simulink model "cable_driven_parallel_robot2022"  (R2022b)
settings: Solver=ode3  StartTime=0.0  StopTime=100  FixedStep=0.01  RelTol=1e-3
values from neighbouring files (symbols this model uses):
  cable_length = 1.2    [Model_Info.m]
  g = 9.81    [Model_Info.m]
  MP_H = 2    [Model_Info.m]
  MP_init_X = 0    [Model_Info.m]
  MP_init_Y = 0    [Model_Info.m]
  MP_init_Z = cable_length + (MP_H/2)    (= 2.2)    [Model_Info.m]
  MP_Ix = (MP_m/12)*(MP_W^2+MP_H^2)    (= 6.66666666667e-05)    [Model_Info.m]
  MP_Iy = (MP_m/12)*(MP_L^2+MP_H^2)    (= 6.66666666667e-05)    [Model_Info.m]
  MP_Iz = (MP_m/12)*(MP_L^2+MP_W^2)    (= 6.66666666667e-05)    [Model_Info.m]
  MP_L = 2    [Model_Info.m]
  MP_m = 0.0001    [Model_Info.m]
  MP_W = 2    [Model_Info.m]
  MR_init_X_L1 = -(MP_L/2)    (= -1)    [Model_Info.m]
  MR_init_X_L2 = (MP_L/2)    (= 1)    [Model_Info.m]
  MR_init_X_L3 = (MP_L/2)    (= 1)    [Model_Info.m]
  MR_init_X_L4 = -(MP_L/2)    (= -1)    [Model_Info.m]
  MR_init_Y_L1 = -(MP_W/2)    (= -1)    [Model_Info.m]
  MR_init_Y_L2 = -(MP_W/2)    (= -1)    [Model_Info.m]
  MR_init_Y_L3 = (MP_W/2)    (= 1)    [Model_Info.m]
  MR_init_Y_L4 = (MP_W/2)    (= 1)    [Model_Info.m]
  MR_init_Yaw_L1 = pi    (= 3.14159265359)    [Model_Info.m]
  MR_init_Yaw_L2 = 0    [Model_Info.m]
  MR_init_Yaw_L3 = 0    [Model_Info.m]
  MR_init_Yaw_L4 = pi    (= 3.14159265359)    [Model_Info.m]
  MR_Jr = (MR_m/12)*(MR_L^2+MR_W^2)    (= 0.333333333333)    [Model_Info.m]
  MR_m = 0.5    [Model_Info.m]
  MR_r = 2    [Model_Info.m]
  MR_WT = 2    [Model_Info.m]
  QR_Ax = 0.25*0    (= 0)    [Model_Info.m]
  QR_Ay = 0.25*0    (= 0)    [Model_Info.m]
  QR_Az = 0.25*0    (= 0)    [Model_Info.m]
  QR_b = 1.14*1e-7    (= 1.14e-07)    [Model_Info.m]
  QR_Ixx = 4.856*1e-3    (= 0.004856)    [Model_Info.m]
  QR_Iyy = 4.856*1e-3    (= 0.004856)    [Model_Info.m]
  QR_Izz = 8.801*1e-3    (= 0.008801)    [Model_Info.m]
  QR_K = 2.980*1e-6    (= 2.98e-06)    [Model_Info.m]
  QR_l = 0.225    [Model_Info.m]
  QR_m = 0.468    [Model_Info.m]
  QR_x0_U1 = -(MP_L/2)    (= -1)    [Model_Info.m]
  QR_x0_U2 = (MP_L/2)    (= 1)    [Model_Info.m]
  QR_x0_U3 = (MP_L/2)    (= 1)    [Model_Info.m]
  QR_x0_U4 = -(MP_L/2)    (= -1)    [Model_Info.m]
  QR_y0_U1 = -(MP_W/2)    (= -1)    [Model_Info.m]
  QR_y0_U2 = -(MP_W/2)    (= -1)    [Model_Info.m]
  QR_y0_U3 = (MP_W/2)    (= 1)    [Model_Info.m]
  QR_y0_U4 = (MP_W/2)    (= 1)    [Model_Info.m]
  QR_z0_U1 = 2*cable_length+(MP_H)    (= 4.4)    [Model_Info.m]
  QR_z0_U2 = 2*cable_length+(MP_H)    (= 4.4)    [Model_Info.m]
  QR_z0_U3 = 2*cable_length+(MP_H)    (= 4.4)    [Model_Info.m]
  QR_z0_U4 = 2*cable_length+(MP_H)    (= 4.4)    [Model_Info.m]
(part 3 of 12)

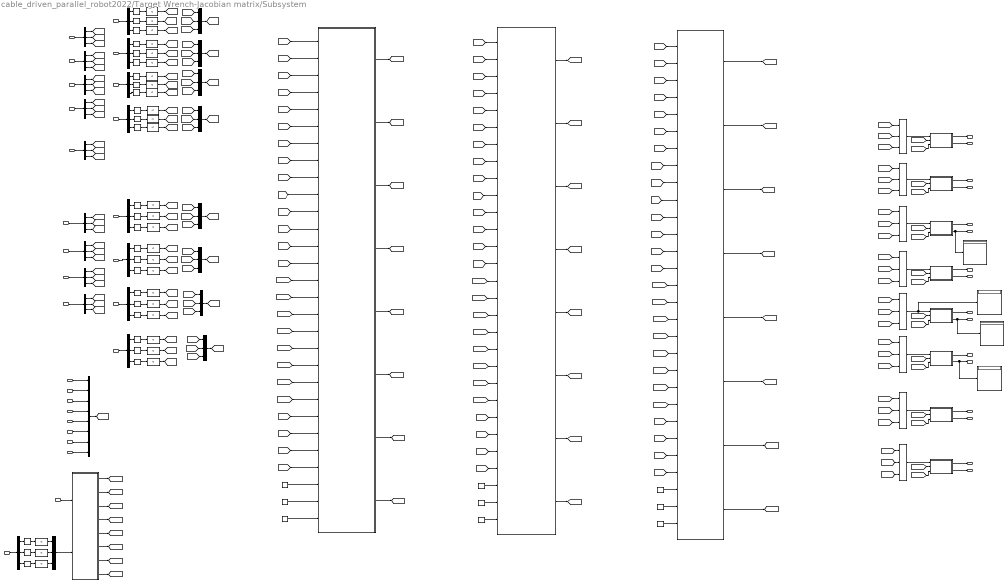
== system cable_driven_parallel_robot2022/Target Wrench-Jacobian matrix/Subsystem ==
  QR_F_U1 : Inport
  QR_F_U2 : Inport  Port=2
  QR_F_U3 : Inport  Port=3
  QR_F_U4 : Inport  Port=4
  MP_F : Inport  Port=5
  MR_F_L1 : Inport  Port=6
  MR_F_L2 : Inport  Port=7
  MR_F_L3 : Inport  Port=8
  MR_F_L4 : Inport  Port=9
  isTension_U1 : Inport  Port=10
  isTension_U2 : Inport  Port=11
  isTension_U3 : Inport  Port=12
  isTension_U4 : Inport  Port=13
  isTension_L1 : Inport  Port=14
  isTension_L2 : Inport  Port=15
  isTension_L3 : Inport  Port=16
  isTension_L4 : Inport  Port=17
  QR_Pose_U1 : Inport  Port=18
  QR_Pose_U2 : Inport  Port=19
  QR_Pose_U3 : Inport  Port=20
  QR_Pose_U4 : Inport  Port=21
  MP_Orientation : Inport  Port=22
  MP_Pose : Inport  Port=23
  MR_Pose_L1 : Inport  Port=24
  MR_Pose_L2 : Inport  Port=25
  MR_Pose_L3 : Inport  Port=26
  MR_Pose_L4 : Inport  Port=27
  Constant : Constant  Value=QR_m
  Constant1 : Constant  Value=MP_m
  Constant2 : Constant  Value=MR_m
  Constant3 : Constant  Value=QR_m
  Constant4 : Constant  Value=MP_m
  Constant5 : Constant  Value=MR_m
  Constant6 : Constant  Value=QR_m
  Constant7 : Constant  Value=MP_m
  Constant8 : Constant  Value=MR_m
  Delay{1..27} (27 alike) : Delay  DelayLength=1
  Demux{,1..17} (18 alike) : Demux  Outputs=3
  Display{,1..3} (4 alike) : Display
  IC1 : InitialCondition  Value=QR_x0_U2
  IC10 : InitialCondition  Value=QR_x0_U4
  IC11 : InitialCondition  Value=QR_y0_U4
  IC12 : InitialCondition  Value=QR_z0_U4
  IC13 : InitialCondition  Value=MR_init_X_L1
  IC14 : InitialCondition  Value=MR_init_Y_L1
  IC{15,18,21,24} (4 alike) : InitialCondition  Value=0
  IC16 : InitialCondition  Value=MR_init_X_L2
  IC17 : InitialCondition  Value=MR_init_Y_L2
  IC19 : InitialCondition  Value=MR_init_X_L3
  IC2 : InitialCondition  Value=QR_y0_U2
  IC20 : InitialCondition  Value=MR_init_Y_L3
  IC22 : InitialCondition  Value=MR_init_X_L4
  IC23 : InitialCondition  Value=MR_init_Y_L4
  IC25 : InitialCondition  Value=MP_init_X
  IC26 : InitialCondition  Value=MP_init_Y
  IC27 : InitialCondition  Value=MP_init_Z
  IC3 : InitialCondition  Value=QR_z0_U2
  IC4 : InitialCondition  Value=QR_x0_U3
  IC5 : InitialCondition  Value=QR_x0_U1
  IC6 : InitialCondition  Value=QR_y0_U1
  IC7 : InitialCondition  Value=QR_z0_U1
  IC8 : InitialCondition  Value=QR_y0_U3
  IC9 : InitialCondition  Value=QR_z0_U3
  MATLAB Function : MATLAB Function  TreatAsAtomicUnit=on
  MATLAB Function1 : MATLAB Function  TreatAsAtomicUnit=on
  MATLAB Function10 : MATLAB Function  TreatAsAtomicUnit=on
  MATLAB Function2 : MATLAB Function  TreatAsAtomicUnit=on
  MATLAB Function3 : MATLAB Function  TreatAsAtomicUnit=on
  MATLAB Function4 : MATLAB Function  TreatAsAtomicUnit=on
  MATLAB Function5 : MATLAB Function  TreatAsAtomicUnit=on
  MATLAB Function6 : MATLAB Function  TreatAsAtomicUnit=on
  MATLAB Function7 : MATLAB Function  TreatAsAtomicUnit=on
  MATLAB Function8 : MATLAB Function  TreatAsAtomicUnit=on
  MATLAB Function9 : MATLAB Function  TreatAsAtomicUnit=on
  Mux : Mux  Inputs=8
  Mux{1..17} (17 alike) : Mux  Inputs=3
  Transformer : Subsystem
  T_MP_U1 : Outport
  T_U1_MP : Outport  Port=2
  T_MP_U2 : Outport  Port=3
  T_U2_MP : Outport  Port=4
  T_MP_U3 : Outport  Port=5
  T_U3_MP : Outport  Port=6
  T_MP_U4 : Outport  Port=7
  T_U4_MP : Outport  Port=8
  T_MP_L1 : Outport  Port=9
  T_L1_MP : Outport  Port=10
  T_MP_L2 : Outport  Port=11
  T_L2_MP : Outport  Port=12
  T_MP_L3 : Outport  Port=13
  T_L3_MP : Outport  Port=14
  T_MP_L4 : Outport  Port=15
  T_L4_MP : Outport  Port=16
  tag scope: isTension=global
  wires:
  Demux/1 -> [QR_Fx_U1]
  Demux/2 -> [QR_Fy_U1]
  Demux/3 -> [QR_Fz_U1]
  Demux1/2 -> [QR_Fy_U2]
  Demux1/1 -> [QR_Fx_U2]
  Demux1/3 -> [QR_Fz_U2]
  Demux2/2 -> [QR_Fy_U3]
  Demux2/1 -> [QR_Fx_U3]
  Demux2/3 -> [QR_Fz_U3]
  Demux3/2 -> [QR_Fy_U4]
  Demux3/1 -> [QR_Fx_U4]
  Demux3/3 -> [QR_Fz_U4]
  Demux4/2 -> [MR_Fy_L1]
  Demux4/1 -> [MR_Fx_L1]
  Demux4/3 -> [MR_Fz_L1]
  Demux5/1 -> [MR_Fx_L2]
  Demux5/3 -> [MR_Fz_L2]
  Demux5/2 -> [MR_Fy_L2]
  Demux6/1 -> [MR_Fx_L3]
  Demux6/3 -> [MR_Fz_L3]
  Demux6/2 -> [MR_Fy_L3]
  Demux7/1 -> [MR_Fx_L4]
  Demux7/3 -> [MR_Fz_L4]
  Demux7/2 -> [MR_Fy_L4]
  Demux8/2 -> [MP_Fy]
  Demux8/3 -> [MP_Fz]
  Demux8/1 -> [MP_Fx]
  QR_F_U1/1 -> Demux/1
  QR_F_U2/1 -> Demux1/1
  QR_F_U3/1 -> Demux2/1
  QR_F_U4/1 -> Demux3/1
  MP_F/1 -> Demux8/1
  MR_F_L2/1 -> Demux5/1
  MR_F_L3/1 -> Demux6/1
  MR_F_L4/1 -> Demux7/1
  MR_F_L1/1 -> Demux4/1
  [QR_Fx_U1] -> MATLAB Function/1(QR_Fx_U1)
  [QR_Fy_U1] -> MATLAB Function1/1(QR_Fy_U1)
  [QR_Fz_U1] -> MATLAB Function2/1(QR_Fz_U1)
  [QR_Fx_U2] -> MATLAB Function/2(QR_Fx_U2)
  [QR_Fx_U3] -> MATLAB Function/3(QR_Fx_U3)
  [QR_Fx_U4] -> MATLAB Function/4(QR_Fx_U4)
  [MP_Fx] -> MATLAB Function/5(MP_Fx)
  [MR_Fx_L1] -> MATLAB Function/6(MR_Fx_L1)
  [MR_Fx_L2] -> MATLAB Function/7(MR_Fx_L2)
  [MR_Fx_L3] -> MATLAB Function/8(MR_Fx_L3)
  [MR_Fx_L4] -> MATLAB Function/9(MR_Fx_L4)
  [QR_Fy_U2] -> MATLAB Function1/2(QR_Fy_U2)
  [QR_Fy_U3] -> MATLAB Function1/3(QR_Fy_U3)
  [QR_Fy_U4] -> MATLAB Function1/4(QR_Fy_U4)
  [MP_Fy] -> MATLAB Function1/5(MP_Fy)
  [MR_Fy_L1] -> MATLAB Function1/6(MR_Fy_L1)
  [MR_Fy_L2] -> MATLAB Function1/7(MR_Fy_L2)
  [MR_Fy_L3] -> MATLAB Function1/8(MR_Fy_L3)
  [MR_Fy_L4] -> MATLAB Function1/9(MR_Fy_L4)
  [QR_Fz_U2] -> MATLAB Function2/2(QR_Fz_U2)
  [QR_Fz_U3] -> MATLAB Function2/3(QR_Fz_U3)
  [QR_Fz_U4] -> MATLAB Function2/4(QR_Fz_U4)
  [MR_Fz_L1] -> MATLAB Function2/6(MR_Fz_L1)
  [MR_Fz_L2] -> MATLAB Function2/7(MR_Fz_L2)
  [MR_Fz_L3] -> MATLAB Function2/8(MR_Fz_L3)
  [MR_Fz_L4] -> MATLAB Function2/9(MR_Fz_L4)
  Mux/1 -> [isTension]
  isTension_U1/1 -> Mux/1
  isTension_U2/1 -> Mux/2
  isTension_U3/1 -> Mux/3
  isTension_U4/1 -> Mux/4
  isTension_L1/1 -> Mux/5
  isTension_L4/1 -> Mux/8
  isTension_L3/1 -> Mux/7
  isTension_L2/1 -> Mux/6
  [isTension] -> MATLAB Function2/10(isTension)
  [isTension] -> MATLAB Function1/10(isTension)
  [isTension] -> MATLAB Function/10(isTension)
  QR_Pose_U1/1 -> Demux9/1
  Demux9/1 -> Delay5/1
  QR_Pose_U2/1 -> Demux10/1
  QR_Pose_U3/1 -> Demux11/1
  QR_Pose_U4/1 -> Demux12/1
  MR_Pose_L1/1 -> Demux14/1
  MR_Pose_L2/1 -> Demux15/1
  MR_Pose_L3/1 -> Demux16/1
  MR_Pose_L4/1 -> Demux17/1
  [QR_X_U1] -> MATLAB Function/11(QR_x_U1)
  [QR_X_U2] -> MATLAB Function/12(QR_x_U2)
  [QR_X_U3] -> MATLAB Function/13(QR_x_U3)
  [QR_X_U4] -> MATLAB Function/14(QR_x_U4)
  [MP_Pose_U1] -> MATLAB Function/15(MP_U1)
  [MR_X_L1] -> MATLAB Function/23(MR_x_L1)
  [MR_X_L2] -> MATLAB Function/24(MR_x_L2)
  [MR_X_L3] -> MATLAB Function/25(MR_x_L3)
  [MR_X_L4] -> MATLAB Function/26(MR_x_L4)
  [QR_Y_U1] -> MATLAB Function1/11(QR_y_U1)
  [QR_Y_U2] -> MATLAB Function1/12(QR_y_U2)
  [QR_Y_U3] -> MATLAB Function1/13(QR_y_U3)
  [QR_Y_U4] -> MATLAB Function1/14(QR_y_U4)
  [MR_Y_L1] -> MATLAB Function1/23(MR_y_L1)
  [MR_Y_L2] -> MATLAB Function1/24(MR_y_L2)
  [MR_Y_L3] -> MATLAB Function1/25(MR_y_L3)
  [MR_Y_L4] -> MATLAB Function1/26(MR_y_L4)
  [QR_Z_U1] -> MATLAB Function2/11(QR_z_U1)
  [QR_Z_U2] -> MATLAB Function2/12(QR_z_U2)
  [QR_Z_U3] -> MATLAB Function2/13(QR_z_U3)
  [QR_Z_U4] -> MATLAB Function2/14(QR_z_U4)
  [MP_Fz] -> MATLAB Function2/5(MP_Fz)
  [MR_Z_L1] -> MATLAB Function2/23(MR_z_L1)
  [MR_Z_L2] -> MATLAB Function2/24(MR_z_L2)
  [MR_Z_L3] -> MATLAB Function2/25(MR_z_L3)
  [MR_Z_L4] -> MATLAB Function2/26(MR_z_L4)
  Constant/1 -> MATLAB Function/27(QR_m)
  Constant1/1 -> MATLAB Function/28(MP_m)
  Constant2/1 -> MATLAB Function/29(MR_m)
  Constant3/1 -> MATLAB Function1/27(QR_m)
  Constant5/1 -> MATLAB Function1/29(MR_m)
  Constant4/1 -> MATLAB Function1/28(MP_m)
  Constant6/1 -> MATLAB Function2/27(QR_m)
  Constant8/1 -> MATLAB Function2/29(MR_m)
  Constant7/1 -> MATLAB Function2/28(MP_m)
  MATLAB Function/1(QR_Tx_U1) -> [QR_Tx_U1]
  MATLAB Function/2(QR_Tx_U2) -> [QR_Tx_U2]
  MATLAB Function/3(QR_Tx_U3) -> [QR_Tx_U3]
  MATLAB Function/4(QR_Tx_U4) -> [QR_Tx_U4]
  MATLAB Function/5(MR_Tx_L1) -> [MR_Tx_L1]
  MATLAB Function/6(MR_Tx_L2) -> [MR_Tx_L2]
  MATLAB Function/7(MR_Tx_L3) -> [MR_Tx_L3]
  MATLAB Function/8(MR_Tx_L4) -> [MR_Tx_L4]
  MATLAB Function1/1(QR_Ty_U1) -> [QR_Ty_U1]
  MATLAB Function1/2(QR_Ty_U2) -> [QR_Ty_U2]
  MATLAB Function1/3(QR_Ty_U3) -> [QR_Ty_U3]
  MATLAB Function1/4(QR_Ty_U4) -> [QR_Ty_U4]
  MATLAB Function1/5(MR_Ty_L1) -> [MR_Ty_L1]
  MATLAB Function1/6(MR_Ty_L2) -> [MR_Ty_L2]
  MATLAB Function1/7(MR_Ty_L3) -> [MR_Ty_L3]
  MATLAB Function1/8(MR_Ty_L4) -> [MR_Ty_L4]
  MATLAB Function2/6(MR_Tz_L2) -> [MR_Tz_L2]
  MATLAB Function2/5(MR_Tz_L1) -> [MR_Tz_L1]
  MATLAB Function2/2(QR_Tz_U2) -> [QR_Tz_U2]
  MATLAB Function2/4(QR_Tz_U4) -> [QR_Tz_U4]
  MATLAB Function2/7(MR_Tz_L3) -> [MR_Tz_L3]
  MATLAB Function2/1(QR_Tz_U1) -> [QR_Tz_U1]
  MATLAB Function2/8(MR_Tz_L4) -> [MR_Tz_L4]
  MATLAB Function2/3(QR_Tz_U3) -> [QR_Tz_U3]
  [QR_Tx_U2] -> Mux1/1
  [QR_Ty_U2] -> Mux1/2
  [QR_Tz_U2] -> Mux1/3
  [QR_Tx_U3] -> Mux2/1
  [QR_Tz_U3] -> Mux2/3
  [QR_Ty_U3] -> Mux2/2
  [QR_Tz_U4] -> Mux3/3
  [QR_Ty_U4] -> Mux3/2
  [QR_Tx_U4] -> Mux3/1
  [MR_Tx_L1] -> Mux4/1
  [MR_Ty_L1] -> Mux4/2
  [MR_Tz_L1] -> Mux4/3
  [MR_Tx_L2] -> Mux5/1
  [MR_Ty_L2] -> Mux5/2
  [MR_Tz_L2] -> Mux5/3
  [MR_Tx_L3] -> Mux6/1
  [MR_Ty_L3] -> Mux6/2
  [MR_Tz_L3] -> Mux6/3
  [MR_Tx_L4] -> Mux7/1
  [MR_Tz_L4] -> Mux7/3
  [MR_Ty_L4] -> Mux7/2
  [QR_Tx_U1] -> Mux8/1
  [QR_Ty_U1] -> Mux8/2
  [QR_Tz_U1] -> Mux8/3
  Mux8/1 -> MATLAB Function3/1(T)
  MP_Orientation/1 -> Transformer/1(MP_Orientation)
  Transformer/1(MP_Pose_U1) -> [MP_Pose_U1]
  Transformer/2(MP_Pose_U2) -> [MP_Pose_U2]
  Transformer/3(MP_Pose_U3) -> [MP_Pose_U3]
  Transformer/4(MP_Pose_U4) -> [MP_Pose_U4]
  Transformer/5(MP_Pose_L1) -> [MP_Pose_L1]
  Transformer/6(MP_Pose_L2) -> [MP_Pose_L2]
  Transformer/7(MP_Pose_L3) -> [MP_Pose_L3]
  Transformer/8(MP_Pose_L4) -> [MP_Pose_L4]
  [MP_Pose_U2] -> MATLAB Function/16(MP_U2)
  [MP_Pose_U3] -> MATLAB Function/17(MP_U3)
  [MP_Pose_U4] -> MATLAB Function/18(MP_U4)
  [MP_Pose_L1] -> MATLAB Function/19(MP_L1)
  [MP_Pose_L2] -> MATLAB Function/20(MP_L2)
  [MP_Pose_L3] -> MATLAB Function/21(MP_L3)
  [MP_Pose_L4] -> MATLAB Function/22(MP_L4)
  [MP_Pose_L2] -> MATLAB Function1/20(MP_L2)
  [MP_Pose_U2] -> MATLAB Function1/16(MP_U2)
  [MP_Pose_U1] -> MATLAB Function1/15(MP_U1)
  [MP_Pose_L1] -> MATLAB Function1/19(MP_L1)
  [MP_Pose_U4] -> MATLAB Function1/18(MP_U4)
  [MP_Pose_L3] -> MATLAB Function1/21(MP_L3)
  [MP_Pose_U3] -> MATLAB Function1/17(MP_U3)
  [MP_Pose_L4] -> MATLAB Function1/22(MP_L4)
  [MP_Pose_U4] -> MATLAB Function2/18(MP_U4)
  [MP_Pose_U1] -> MATLAB Function2/15(MP_U1)
  [MP_Pose_L2] -> MATLAB Function2/20(MP_L2)
  [MP_Pose_L3] -> MATLAB Function2/21(MP_L3)
  [MP_Pose_U2] -> MATLAB Function2/16(MP_U2)
  [MP_Pose_L1] -> MATLAB Function2/19(MP_L1)
  [MP_Pose_L4] -> MATLAB Function2/22(MP_L4)
  [MP_Pose_U3] -> MATLAB Function2/17(MP_U3)
  Delay5/1 -> IC5/1
  Delay6/1 -> IC6/1
  IC5/1 -> [QR_X_U1]
  IC6/1 -> [QR_Y_U1]
  Demux9/2 -> Delay6/1
  Delay7/1 -> IC7/1
  Demux9/3 -> Delay7/1
  IC7/1 -> [QR_Z_U1]
  Demux10/1 -> Delay8/1
  Demux10/2 -> Delay1/1
  Demux10/3 -> Delay2/1
  Demux11/1 -> Delay3/1
  Demux11/2 -> Delay4/1
  Demux11/3 -> Delay9/1
  Demux12/1 -> Delay10/1
  Demux12/2 -> Delay11/1
  Demux12/3 -> Delay12/1
  Delay14/1 -> IC14/1
  Demux14/2 -> Delay14/1
  Delay13/1 -> IC13/1
  IC14/1 -> [MR_Y_L1]
  Delay15/1 -> IC15/1
  Demux14/3 -> Delay15/1
  IC13/1 -> [MR_X_L1]
  IC15/1 -> [MR_Z_L1]
  Demux14/1 -> Delay13/1
  Demux16/3 -> Delay18/1
  Demux16/1 -> Delay16/1
  Demux16/2 -> Delay17/1
  Demux15/3 -> Delay21/1
  Demux15/1 -> Delay19/1
  Demux15/2 -> Delay20/1
  Demux17/3 -> Delay24/1
  Demux17/1 -> Delay22/1
  Demux17/2 -> Delay23/1
  IC2/1 -> [QR_Y_U2]
  Delay1/1 -> IC2/1
  Delay8/1 -> IC1/1
  Delay2/1 -> IC3/1
  IC3/1 -> [QR_Z_U2]
  IC1/1 -> [QR_X_U2]
  IC8/1 -> [QR_Y_U3]
  Delay4/1 -> IC8/1
  Delay3/1 -> IC4/1
  Delay9/1 -> IC9/1
  IC9/1 -> [QR_Z_U3]
  IC4/1 -> [QR_X_U3]
  IC11/1 -> [QR_Y_U4]
  Delay11/1 -> IC11/1
  Delay10/1 -> IC10/1
  Delay12/1 -> IC12/1
  IC12/1 -> [QR_Z_U4]
  IC10/1 -> [QR_X_U4]
  Delay20/1 -> IC17/1
  IC17/1 -> [MR_Y_L2]
  IC18/1 -> [MR_Z_L2]
  Delay21/1 -> IC18/1
  Delay19/1 -> IC16/1
  IC16/1 -> [MR_X_L2]
  Delay17/1 -> IC20/1
  IC20/1 -> [MR_Y_L3]
  IC21/1 -> [MR_Z_L3]
  Delay18/1 -> IC21/1
  Delay16/1 -> IC19/1
  IC19/1 -> [MR_X_L3]
  Delay23/1 -> IC23/1
  IC23/1 -> [MR_Y_L4]
  IC24/1 -> [MR_Z_L4]
  Delay24/1 -> IC24/1
  Delay22/1 -> IC22/1
  IC22/1 -> [MR_X_L4]
  MP_Pose/1 -> Demux13/1
  Delay25/1 -> IC25/1
  IC25/1 -> Mux9/1
  Delay27/1 -> IC27/1
  Delay26/1 -> IC26/1
  IC27/1 -> Mux9/3
  IC26/1 -> Mux9/2
  Demux13/3 -> Delay27/1
  Demux13/1 -> Delay25/1
  Demux13/2 -> Delay26/1
  Mux9/1 -> Transformer/2(MP_Pose)
  MATLAB Function3/1(T_MP) -> T_MP_U1/1
  MATLAB Function3/2(T_ME) -> T_U1_MP/1
  [MP_Pose_U1] -> MATLAB Function3/2(MP_Pose)
  [QR_Pose_U1] -> MATLAB Function3/3(ME_Pose)
  [QR_X_U1] -> Mux10/1
  [QR_Y_U1] -> Mux10/2
  [QR_Z_U1] -> Mux10/3
  Mux10/1 -> [QR_Pose_U1]
  [QR_X_U2] -> Mux11/1
  Mux11/1 -> [QR_Pose_U2]
  [QR_Z_U2] -> Mux11/3
  [QR_Y_U2] -> Mux11/2
  [QR_Z_U3] -> Mux12/3
  [QR_Y_U3] -> Mux12/2
  Mux12/1 -> [QR_Pose_U3]
  [QR_X_U3] -> Mux12/1
  [QR_Z_U4] -> Mux13/3
  [QR_Y_U4] -> Mux13/2
  Mux13/1 -> [QR_Pose_U4]
  [QR_X_U4] -> Mux13/1
  [MR_Z_L1] -> Mux14/3
  [MR_Y_L1] -> Mux14/2
  [MR_X_L1] -> Mux14/1
  Mux14/1 -> [MR_Pose_L1]
  Mux15/1 -> [MR_Pose_L2]
  [MR_X_L2] -> Mux15/1
  [MR_Z_L2] -> Mux15/3
  [MR_Y_L2] -> Mux15/2
  [MR_Z_L3] -> Mux16/3
  [MR_X_L3] -> Mux16/1
  [MR_Y_L3] -> Mux16/2
  Mux16/1 -> [MR_Pose_L3]
  [MR_Z_L4] -> Mux17/3
  [MR_X_L4] -> Mux17/1
  [MR_Y_L4] -> Mux17/2
  Mux17/1 -> [MR_Pose_L4]
  [QR_Pose_U2] -> MATLAB Function4/3(ME_Pose)
  MATLAB Function4/2(T_ME) -> T_U2_MP/1
  [MP_Pose_U2] -> MATLAB Function4/2(MP_Pose)
  MATLAB Function4/1(T_MP) -> T_MP_U2/1
  Mux1/1 -> MATLAB Function4/1(T)
  MATLAB Function5/1(T_MP) -> T_MP_U3/1
  Mux2/1 -> MATLAB Function5/1(T)
  [QR_Pose_U3] -> MATLAB Function5/3(ME_Pose)
  [MP_Pose_U3] -> MATLAB Function5/2(MP_Pose)
  Mux3/1 -> MATLAB Function6/1(T)
  [MP_Pose_U4] -> MATLAB Function6/2(MP_Pose)
  MATLAB Function6/2(T_ME) -> T_U4_MP/1
  [QR_Pose_U4] -> MATLAB Function6/3(ME_Pose)
  MATLAB Function6/1(T_MP) -> T_MP_U4/1
  [MR_Pose_L1] -> MATLAB Function7/3(ME_Pose)
  MATLAB Function7/1(T_MP) -> T_MP_L1/1
  MATLAB Function7/2(T_ME) -> Display1/1, T_L1_MP/1
  [MP_Pose_L1] -> MATLAB Function7/2(MP_Pose)
  MATLAB Function8/1(T_MP) -> T_MP_L2/1
  [MP_Pose_L2] -> MATLAB Function8/2(MP_Pose)
  [MR_Pose_L2] -> MATLAB Function8/3(ME_Pose)
  Mux5/1 -> MATLAB Function8/1(T)
  Mux6/1 -> MATLAB Function9/1(T)
  MATLAB Function9/2(T_ME) -> T_L3_MP/1
  [MR_Pose_L3] -> MATLAB Function9/3(ME_Pose)
  [MP_Pose_L3] -> MATLAB Function9/2(MP_Pose)
  MATLAB Function9/1(T_MP) -> T_MP_L3/1
  Mux7/1 -> MATLAB Function10/1(T)
  [MP_Pose_L4] -> MATLAB Function10/2(MP_Pose)
  [MR_Pose_L4] -> MATLAB Function10/3(ME_Pose)
  MATLAB Function10/2(T_ME) -> T_L4_MP/1
  MATLAB Function10/1(T_MP) -> T_MP_L4/1
  MATLAB Function5/2(T_ME) -> Display/1, T_U3_MP/1
  MATLAB Function8/2(T_ME) -> Display2/1, T_L2_MP/1
  Mux4/1 -> Display3/1, MATLAB Function7/1(T)

== system cable_driven_parallel_robot2022/Actuators-CableTension-MovingPlatform/2 Wheels Diffrential Mobile Robot/2 Wheels Diffrential Mobile Robot ==
  TR : Inport
  TL : Inport  Port=2
  Tx : Inport  Port=3
  Ty : Inport  Port=4
  Tz : Inport  Port=5
  Jr : Inport  Port=6
  mass : Inport  Port=7
  r : Inport  Port=8
  Wheel Track : Inport  Port=9
  2 Wheels Diffrential Mobile Robot : MATLAB Function  TreatAsAtomicUnit=on
  2 Wheels Diffrential Mobile Robot Transformation to Global : MATLAB Function  TreatAsAtomicUnit=on
  Delay{,1..3} (4 alike) : Delay  DelayLength=1
  Derivative1 : Derivative
  Derivative2 : Derivative
  Derivative3 : Derivative
  Integrator1 : Integrator
  Integrator2 : Integrator
  Integrator3 : Integrator  InitialCondition=MR_init_X_L1
  Integrator4 : Integrator  ExternalReset=rising
  Integrator5 : Integrator  InitialCondition=MR_init_Yaw_L1
  Integrator6 : Integrator
  Integrator7 : Integrator  InitialCondition=MR_init_Y_L1
  Integrator8 : Integrator  ExternalReset=rising
  Vel_Manager : Subsystem
  wrap angle (Rad) : Subsystem
  X : Outport
  Vx : Outport  Port=2
  ax : Outport  Port=3
  Y : Outport  Port=4
  Vy : Outport  Port=5
  ay : Outport  Port=6
  Z : Outport  Port=7
  Vz : Outport  Port=8
  az : Outport  Port=9
  yaw : Outport  Port=10
  yaw_dot : Outport  Port=11
  wires:
  Integrator8/1 -> [Z], Z/1
  2 Wheels Diffrential Mobile Robot/1(ax) -> Integrator1/1
  Tz/1 -> 2 Wheels Diffrential Mobile Robot/5(Tz)
  2 Wheels Diffrential Mobile Robot/4(alpha_r) -> Integrator2/1
  Integrator2/1 -> yaw_dot/1, Integrator5/1
  2 Wheels Diffrential Mobile Robot/3(az) -> Integrator4/1
  2 Wheels Diffrential Mobile Robot Transformation to Global/1(Vbx) -> Integrator3/1, Derivative1/1, Vx/1
  Tx/1 -> 2 Wheels Diffrential Mobile Robot/3(Tx)
  wrap angle (Rad)/1(angle_out) -> yaw/1, 2 Wheels Diffrential Mobile Robot Transformation to Global/4(yaw)
  2 Wheels Diffrential Mobile Robot Transformation to Global/3(Vbz) -> Integrator8/1, Vz/1, Derivative2/1
  Integrator1/1 -> 2 Wheels Diffrential Mobile Robot Transformation to Global/1(Vx)
  Wheel Track/1 -> 2 Wheels Diffrential Mobile Robot/9(WT)
  Jr/1 -> 2 Wheels Diffrential Mobile Robot/6(Jr)
  Integrator4/1 -> 2 Wheels Diffrential Mobile Robot Transformation to Global/3(Vz)
  TR/1 -> 2 Wheels Diffrential Mobile Robot/1(TR)
  TL/1 -> 2 Wheels Diffrential Mobile Robot/2(TL)
  r/1 -> 2 Wheels Diffrential Mobile Robot/8(r)
  Integrator3/1 -> X/1
  mass/1 -> 2 Wheels Diffrential Mobile Robot/7(mr)
  Derivative1/1 -> ax/1
  Derivative2/1 -> az/1
  Integrator5/1 -> wrap angle (Rad)/1(angle_in)
  2 Wheels Diffrential Mobile Robot Transformation to Global/2(Vby) -> Integrator7/1, Vy/1, Derivative3/1
  Integrator7/1 -> Y/1
  Derivative3/1 -> ay/1
  [rest] -> Integrator4/2
  [rest] -> Integrator8/2
  Ty/1 -> 2 Wheels Diffrential Mobile Robot/4(Ty)
  2 Wheels Diffrential Mobile Robot/2(ay) -> Integrator6/1
  Integrator6/1 -> 2 Wheels Diffrential Mobile Robot Transformation to Global/2(Vy)
  Vel_Manager/4(Reste) -> [Reste]
  Vel_Manager/2(Vy_min) -> [Vy_min]
  Vel_Manager/1(Vx_min) -> [Vx_min]
  Vel_Manager/3(Vz_min) -> [Vz_min]
  [Vx_min] -> Delay1/1
  [Vy_min] -> Delay2/1
  [Vz_min] -> Delay3/1
  [Reste] -> 2 Wheels Diffrential Mobile Robot Transformation to Global/8(reste)
  Delay1/1 -> 2 Wheels Diffrential Mobile Robot Transformation to Global/5(Vx_min)
  Delay2/1 -> 2 Wheels Diffrential Mobile Robot Transformation to Global/6(Vy_min)
  Delay3/1 -> 2 Wheels Diffrential Mobile Robot Transformation to Global/7(Vz_min)
  Delay/1 -> 2 Wheels Diffrential Mobile Robot Transformation to Global/9(z)
  [Z] -> Delay/1
  2 Wheels Diffrential Mobile Robot Transformation to Global/4(rest) -> [rest]

== system cable_driven_parallel_robot2022/Actuators-CableTension-MovingPlatform/2 Wheels Diffrential Mobile Robot1/2 Wheels Diffrential Mobile Robot ==
  TR : Inport
  TL : Inport  Port=2
  Tx : Inport  Port=3
  Ty : Inport  Port=4
  Tz : Inport  Port=5
  Jr : Inport  Port=6
  mass : Inport  Port=7
  r : Inport  Port=8
  Wheel Track : Inport  Port=9
  2 Wheels Diffrential Mobile Robot : MATLAB Function  TreatAsAtomicUnit=on
  2 Wheels Diffrential Mobile Robot Transformation to Global : MATLAB Function  TreatAsAtomicUnit=on
  Delay{,1..3} (4 alike) : Delay  DelayLength=1
  Derivative1 : Derivative
  Derivative2 : Derivative
  Derivative3 : Derivative
  Integrator1 : Integrator
  Integrator2 : Integrator
  Integrator3 : Integrator  InitialCondition=MR_init_X_L2
  Integrator4 : Integrator  ExternalReset=rising
  Integrator5 : Integrator  InitialCondition=MR_init_Yaw_L2
  Integrator6 : Integrator
  Integrator7 : Integrator  InitialCondition=MR_init_Y_L2
  Integrator8 : Integrator  ExternalReset=rising
  Vel_Manager : Subsystem
  wrap angle (Rad) : Subsystem
  X : Outport
  Vx : Outport  Port=2
  ax : Outport  Port=3
  Y : Outport  Port=4
  Vy : Outport  Port=5
  ay : Outport  Port=6
  Z : Outport  Port=7
  Vz : Outport  Port=8
  az : Outport  Port=9
  yaw : Outport  Port=10
  yaw_dot : Outport  Port=11
  wires:
  Integrator6/1 -> 2 Wheels Diffrential Mobile Robot Transformation to Global/2(Vy)
  2 Wheels Diffrential Mobile Robot/2(ay) -> Integrator6/1
  Ty/1 -> 2 Wheels Diffrential Mobile Robot/4(Ty)
  [rest] -> Integrator8/2
  [rest] -> Integrator4/2
  Derivative3/1 -> ay/1
  Integrator7/1 -> Y/1
  2 Wheels Diffrential Mobile Robot Transformation to Global/2(Vby) -> Integrator7/1, Vy/1, Derivative3/1
  Integrator5/1 -> wrap angle (Rad)/1(angle_in)
  Derivative2/1 -> az/1
  Derivative1/1 -> ax/1
  mass/1 -> 2 Wheels Diffrential Mobile Robot/7(mr)
  Integrator3/1 -> X/1
  r/1 -> 2 Wheels Diffrential Mobile Robot/8(r)
  TL/1 -> 2 Wheels Diffrential Mobile Robot/2(TL)
  TR/1 -> 2 Wheels Diffrential Mobile Robot/1(TR)
  Integrator4/1 -> 2 Wheels Diffrential Mobile Robot Transformation to Global/3(Vz)
  Jr/1 -> 2 Wheels Diffrential Mobile Robot/6(Jr)
  Wheel Track/1 -> 2 Wheels Diffrential Mobile Robot/9(WT)
  Integrator1/1 -> 2 Wheels Diffrential Mobile Robot Transformation to Global/1(Vx)
  2 Wheels Diffrential Mobile Robot Transformation to Global/3(Vbz) -> Integrator8/1, Vz/1, Derivative2/1
  wrap angle (Rad)/1(angle_out) -> yaw/1, 2 Wheels Diffrential Mobile Robot Transformation to Global/4(yaw)
  Tx/1 -> 2 Wheels Diffrential Mobile Robot/3(Tx)
  2 Wheels Diffrential Mobile Robot Transformation to Global/1(Vbx) -> Integrator3/1, Vx/1, Derivative1/1
  2 Wheels Diffrential Mobile Robot/3(az) -> Integrator4/1
  Integrator2/1 -> Integrator5/1, yaw_dot/1
  2 Wheels Diffrential Mobile Robot/4(alpha_r) -> Integrator2/1
  Tz/1 -> 2 Wheels Diffrential Mobile Robot/5(Tz)
  2 Wheels Diffrential Mobile Robot Transformation to Global/4(rest) -> [rest]
  2 Wheels Diffrential Mobile Robot/1(ax) -> Integrator1/1
  Integrator8/1 -> Z/1, [Z]
  Vel_Manager/1(Vx_min) -> [Vx_min]
  Vel_Manager/3(Vz_min) -> [Vz_min]
  Vel_Manager/2(Vy_min) -> [Vy_min]
  Vel_Manager/4(Reste) -> [Reste]
  [Vx_min] -> Delay3/1
  [Vy_min] -> Delay2/1
  [Vz_min] -> Delay1/1
  [Reste] -> 2 Wheels Diffrential Mobile Robot Transformation to Global/8(reste)
  Delay1/1 -> 2 Wheels Diffrential Mobile Robot Transformation to Global/7(Vz_min)
  Delay2/1 -> 2 Wheels Diffrential Mobile Robot Transformation to Global/6(Vy_min)
  Delay3/1 -> 2 Wheels Diffrential Mobile Robot Transformation to Global/5(Vx_min)
  [Z] -> Delay/1
  Delay/1 -> 2 Wheels Diffrential Mobile Robot Transformation to Global/9(z)

== system cable_driven_parallel_robot2022/Actuators-CableTension-MovingPlatform/2 Wheels Diffrential Mobile Robot2/2 Wheels Diffrential Mobile Robot ==
  TR : Inport
  TL : Inport  Port=2
  Tx : Inport  Port=3
  Ty : Inport  Port=4
  Tz : Inport  Port=5
  Jr : Inport  Port=6
  mass : Inport  Port=7
  r : Inport  Port=8
  Wheel Track : Inport  Port=9
  2 Wheels Diffrential Mobile Robot : MATLAB Function  TreatAsAtomicUnit=on
  2 Wheels Diffrential Mobile Robot Transformation to Global : MATLAB Function  TreatAsAtomicUnit=on
  Delay{,1..3} (4 alike) : Delay  DelayLength=1
  Derivative1 : Derivative
  Derivative2 : Derivative
  Derivative3 : Derivative
  Integrator1 : Integrator
  Integrator2 : Integrator
  Integrator3 : Integrator  InitialCondition=MR_init_X_L3
  Integrator4 : Integrator  ExternalReset=rising
  Integrator5 : Integrator  InitialCondition=MR_init_Yaw_L3
  Integrator6 : Integrator
  Integrator7 : Integrator  InitialCondition=MR_init_Y_L3
  Integrator8 : Integrator  ExternalReset=rising
  Vel_Manager : Subsystem
  wrap angle (Rad) : Subsystem
  X : Outport
  Vx : Outport  Port=2
  ax : Outport  Port=3
  Y : Outport  Port=4
  Vy : Outport  Port=5
  ay : Outport  Port=6
  Z : Outport  Port=7
  Vz : Outport  Port=8
  az : Outport  Port=9
  yaw : Outport  Port=10
  yaw_dot : Outport  Port=11
  wires:
  Integrator6/1 -> 2 Wheels Diffrential Mobile Robot Transformation to Global/2(Vy)
  2 Wheels Diffrential Mobile Robot/2(ay) -> Integrator6/1
  Ty/1 -> 2 Wheels Diffrential Mobile Robot/4(Ty)
  [rest] -> Integrator8/2
  [rest] -> Integrator4/2
  Derivative3/1 -> ay/1
  Integrator7/1 -> Y/1
  2 Wheels Diffrential Mobile Robot Transformation to Global/2(Vby) -> Derivative3/1, Vy/1, Integrator7/1
  Delay/1 -> 2 Wheels Diffrential Mobile Robot Transformation to Global/9(z)
  [Z] -> Delay/1
  Integrator5/1 -> wrap angle (Rad)/1(angle_in)
  Derivative2/1 -> az/1
  Derivative1/1 -> ax/1
  mass/1 -> 2 Wheels Diffrential Mobile Robot/7(mr)
  Integrator3/1 -> X/1
  r/1 -> 2 Wheels Diffrential Mobile Robot/8(r)
  TL/1 -> 2 Wheels Diffrential Mobile Robot/2(TL)
  TR/1 -> 2 Wheels Diffrential Mobile Robot/1(TR)
  Integrator4/1 -> 2 Wheels Diffrential Mobile Robot Transformation to Global/3(Vz)
  Jr/1 -> 2 Wheels Diffrential Mobile Robot/6(Jr)
  Wheel Track/1 -> 2 Wheels Diffrential Mobile Robot/9(WT)
  Integrator1/1 -> 2 Wheels Diffrential Mobile Robot Transformation to Global/1(Vx)
  2 Wheels Diffrential Mobile Robot Transformation to Global/3(Vbz) -> Integrator8/1, Vz/1, Derivative2/1
  wrap angle (Rad)/1(angle_out) -> yaw/1, 2 Wheels Diffrential Mobile Robot Transformation to Global/4(yaw)
  Tx/1 -> 2 Wheels Diffrential Mobile Robot/3(Tx)
  2 Wheels Diffrential Mobile Robot Transformation to Global/1(Vbx) -> Derivative1/1, Integrator3/1, Vx/1
  2 Wheels Diffrential Mobile Robot/3(az) -> Integrator4/1
  Integrator2/1 -> Integrator5/1, yaw_dot/1
  2 Wheels Diffrential Mobile Robot/4(alpha_r) -> Integrator2/1
  Tz/1 -> 2 Wheels Diffrential Mobile Robot/5(Tz)
  2 Wheels Diffrential Mobile Robot Transformation to Global/4(rest) -> [rest]
  2 Wheels Diffrential Mobile Robot/1(ax) -> Integrator1/1
  Integrator8/1 -> Z/1, [Z]
  Vel_Manager/2(Vy_min) -> [Vy_min]
  Vel_Manager/4(Reste) -> [Reste]
  Vel_Manager/3(Vz_min) -> [Vz_min]
  Vel_Manager/1(Vx_min) -> [Vx_min]
  [Vy_min] -> Delay2/1
  [Vx_min] -> Delay3/1
  [Vz_min] -> Delay1/1
  [Reste] -> 2 Wheels Diffrential Mobile Robot Transformation to Global/8(reste)
  Delay1/1 -> 2 Wheels Diffrential Mobile Robot Transformation to Global/7(Vz_min)
  Delay2/1 -> 2 Wheels Diffrential Mobile Robot Transformation to Global/6(Vy_min)
  Delay3/1 -> 2 Wheels Diffrential Mobile Robot Transformation to Global/5(Vx_min)

== system cable_driven_parallel_robot2022/Actuators-CableTension-MovingPlatform/2 Wheels Diffrential Mobile Robot3/2 Wheels Diffrential Mobile Robot ==
  TR : Inport
  TL : Inport  Port=2
  Tx : Inport  Port=3
  Ty : Inport  Port=4
  Tz : Inport  Port=5
  Jr : Inport  Port=6
  mass : Inport  Port=7
  r : Inport  Port=8
  Wheel Track : Inport  Port=9
  2 Wheels Diffrential Mobile Robot : MATLAB Function  TreatAsAtomicUnit=on
  2 Wheels Diffrential Mobile Robot Transformation to Global : MATLAB Function  TreatAsAtomicUnit=on
  Delay{,1..3} (4 alike) : Delay  DelayLength=1
  Derivative1 : Derivative
  Derivative2 : Derivative
  Derivative3 : Derivative
  Integrator1 : Integrator
  Integrator2 : Integrator
  Integrator3 : Integrator  InitialCondition=MR_init_X_L4
  Integrator4 : Integrator  ExternalReset=rising
  Integrator5 : Integrator  InitialCondition=MR_init_Yaw_L4
  Integrator6 : Integrator
  Integrator7 : Integrator  InitialCondition=MR_init_Y_L4
  Integrator8 : Integrator  ExternalReset=rising
  Vel_Manager : Subsystem
  wrap angle (Rad) : Subsystem
  X : Outport
  Vx : Outport  Port=2
  ax : Outport  Port=3
  Y : Outport  Port=4
  Vy : Outport  Port=5
  ay : Outport  Port=6
  Z : Outport  Port=7
  Vz : Outport  Port=8
  az : Outport  Port=9
  yaw : Outport  Port=10
  yaw_dot : Outport  Port=11
  wires:
  Integrator6/1 -> 2 Wheels Diffrential Mobile Robot Transformation to Global/2(Vy)
  2 Wheels Diffrential Mobile Robot/2(ay) -> Integrator6/1
  Ty/1 -> 2 Wheels Diffrential Mobile Robot/4(Ty)
  [rest] -> Integrator8/2
  [rest] -> Integrator4/2
  Derivative3/1 -> ay/1
  Integrator7/1 -> Y/1
  2 Wheels Diffrential Mobile Robot Transformation to Global/2(Vby) -> Integrator7/1, Vy/1, Derivative3/1
  Delay/1 -> 2 Wheels Diffrential Mobile Robot Transformation to Global/9(z)
  [Z] -> Delay/1
  Integrator5/1 -> wrap angle (Rad)/1(angle_in)
  Derivative2/1 -> az/1
  Derivative1/1 -> ax/1
  mass/1 -> 2 Wheels Diffrential Mobile Robot/7(mr)
  Integrator3/1 -> X/1
  r/1 -> 2 Wheels Diffrential Mobile Robot/8(r)
  TL/1 -> 2 Wheels Diffrential Mobile Robot/2(TL)
  TR/1 -> 2 Wheels Diffrential Mobile Robot/1(TR)
  Integrator4/1 -> 2 Wheels Diffrential Mobile Robot Transformation to Global/3(Vz)
  Jr/1 -> 2 Wheels Diffrential Mobile Robot/6(Jr)
  Wheel Track/1 -> 2 Wheels Diffrential Mobile Robot/9(WT)
  Integrator1/1 -> 2 Wheels Diffrential Mobile Robot Transformation to Global/1(Vx)
  2 Wheels Diffrential Mobile Robot Transformation to Global/3(Vbz) -> Integrator8/1, Vz/1, Derivative2/1
  wrap angle (Rad)/1(angle_out) -> yaw/1, 2 Wheels Diffrential Mobile Robot Transformation to Global/4(yaw)
  Tx/1 -> 2 Wheels Diffrential Mobile Robot/3(Tx)
  2 Wheels Diffrential Mobile Robot Transformation to Global/1(Vbx) -> Derivative1/1, Integrator3/1, Vx/1
  2 Wheels Diffrential Mobile Robot/3(az) -> Integrator4/1
  Integrator2/1 -> Integrator5/1, yaw_dot/1
  2 Wheels Diffrential Mobile Robot/4(alpha_r) -> Integrator2/1
  Tz/1 -> 2 Wheels Diffrential Mobile Robot/5(Tz)
  2 Wheels Diffrential Mobile Robot Transformation to Global/4(rest) -> [rest]
  2 Wheels Diffrential Mobile Robot/1(ax) -> Integrator1/1
  Integrator8/1 -> Z/1, [Z]
  Vel_Manager/4(Reste) -> [Reste]
  Vel_Manager/1(Vx_min) -> [Vx_min]
  Vel_Manager/3(Vz_min) -> [Vz_min]
  Vel_Manager/2(Vy_min) -> [Vy_min]
  [Vx_min] -> Delay1/1
  [Vy_min] -> Delay2/1
  [Vz_min] -> Delay3/1
  [Reste] -> 2 Wheels Diffrential Mobile Robot Transformation to Global/8(reste)
  Delay1/1 -> 2 Wheels Diffrential Mobile Robot Transformation to Global/5(Vx_min)
  Delay2/1 -> 2 Wheels Diffrential Mobile Robot Transformation to Global/6(Vy_min)
  Delay3/1 -> 2 Wheels Diffrential Mobile Robot Transformation to Global/7(Vz_min)

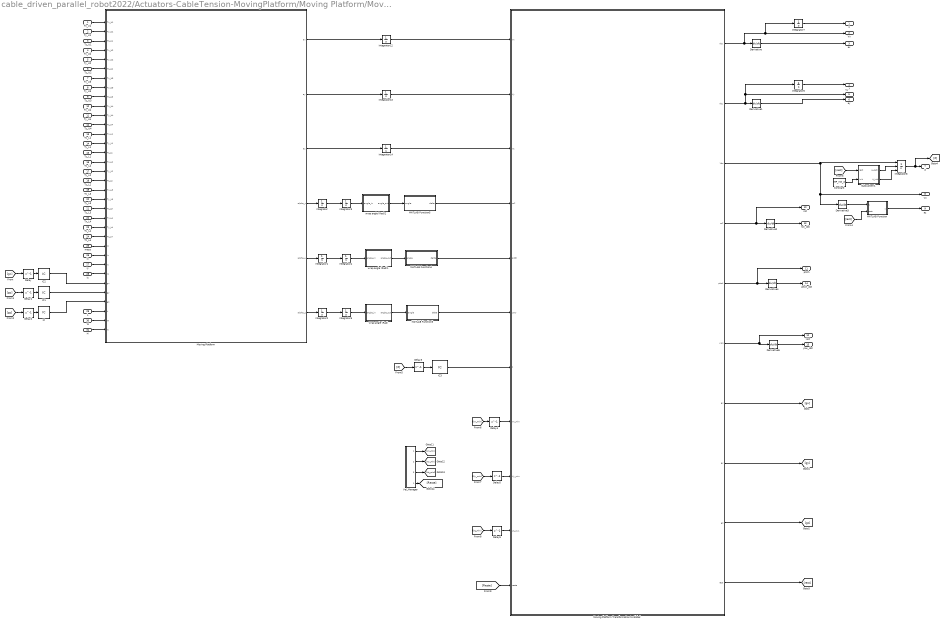
== system cable_driven_parallel_robot2022/Actuators-CableTension-MovingPlatform/Moving Platform/Moving Platform ==
  Tx_U1 : Inport
  Ty_U1 : Inport  Port=2
  Tz_U1 : Inport  Port=3
  Tx_U2 : Inport  Port=4
  Ty_U2 : Inport  Port=5
  Tz_U2 : Inport  Port=6
  Tx_U3 : Inport  Port=7
  Ty_U3 : Inport  Port=8
  Tz_U3 : Inport  Port=9
  Tx_U4 : Inport  Port=10
  Ty_U4 : Inport  Port=11
  Tz_U4 : Inport  Port=12
  Tx_L1 : Inport  Port=13
  Ty_L1 : Inport  Port=14
  Tz_L1 : Inport  Port=15
  Tx_L2 : Inport  Port=16
  Ty_L2 : Inport  Port=17
  Tz_L2 : Inport  Port=18
  Tx_L3 : Inport  Port=19
  Ty_L3 : Inport  Port=20
  Tz_L3 : Inport  Port=21
  Tx_L4 : Inport  Port=22
  Ty_L4 : Inport  Port=23
  Tz_L4 : Inport  Port=24
  mass : Inport  Port=25
  Ix : Inport  Port=26
  Iy : Inport  Port=27
  Iz : Inport  Port=28
  L : Inport  Port=29
  W : Inport  Port=30
  H : Inport  Port=31
  Constant : Constant  Value=MP_init_Z
  Delay{,1..6} (7 alike) : Delay  DelayLength=1
  Derivative{,1..5} (6 alike) : Derivative
  IC : InitialCondition  Value=9.81
  IC1 : InitialCondition  Value=0
  IC2 : InitialCondition  Value=0
  IC3 : InitialCondition  Value=MP_init_Z
  Integrator{,1..5,12..14} (9 alike) : Integrator
  Integrator6 : Integrator  InitialCondition=MP_init_Y
  Integrator7 : Integrator  InitialCondition=MP_init_X
  Integrator8 : Integrator  ExternalReset=rising  InitialConditionSource=external
  MATLAB Function : MATLAB Function  TreatAsAtomicUnit=on
  MATLAB Function3 : MATLAB Function  TreatAsAtomicUnit=on
  MATLAB Function4 : MATLAB Function  TreatAsAtomicUnit=on
  MATLAB Function5 : MATLAB Function  TreatAsAtomicUnit=on
  Moving Platform : MATLAB Function  TreatAsAtomicUnit=on
  Moving Platform Transformation to Global : MATLAB Function  TreatAsAtomicUnit=on
  Subsystem1 : Subsystem
  Vel_Manager : Subsystem
  wrap angle (Rad) : Subsystem
  wrap angle (Rad)1 : Subsystem
  wrap angle (Rad)2 : Subsystem
  X : Outport
  Vx : Outport  Port=2
  ax : Outport  Port=3
  Y : Outport  Port=4
  Vy : Outport  Port=5
  ay : Outport  Port=6
  Z : Outport  Port=7
  Vz : Outport  Port=8
  az : Outport  Port=9
  roll : Outport  Port=10
  pitch : Outport  Port=11
  yaw : Outport  Port=12
  roll_dot : Outport  Port=13
  pitch_dot : Outport  Port=14
  yaw_dot : Outport  Port=15
  wires:
  Tx_U3/1 -> Moving Platform/7(Tx_U3)
  Moving Platform/6(alpha_z) -> Integrator2/1
  Tz_U4/1 -> Moving Platform/12(Tz_U4)
  Integrator2/1 -> Integrator5/1
  Moving Platform Transformation to Global/4(roll) -> roll/1, Derivative2/1
  Tz_L4/1 -> Moving Platform/24(Tz_L4)
  Moving Platform/2(ay) -> Integrator13/1
  Moving Platform Transformation to Global/1(Vbx) -> Derivative/1, Vx/1, Integrator7/1
  MATLAB Function3/1(delta) -> Moving Platform Transformation to Global/6("yaw ")
  Integrator5/1 -> wrap angle (Rad)/1(angle_in)
  MATLAB Function4/1(delta) -> Moving Platform Transformation to Global/5("pitch ")
  Integrator1/1 -> Integrator4/1
  Tz_U1/1 -> Moving Platform/3(Tz_U1)
  Integrator4/1 -> wrap angle (Rad)1/1(angle_in)
  Ty_L3/1 -> Moving Platform/20(Ty_L3)
  wrap angle (Rad)2/1(angle_out) -> MATLAB Function5/1(angle)
  W/1 -> Moving Platform/33(W)
  Moving Platform/4(alpha_x) -> Integrator/1
  Moving Platform Transformation to Global/6(yaw) -> Derivative5/1, yaw/1
  Integrator6/1 -> Y/1
  Tx_L2/1 -> Moving Platform/16(Tx_L2)
  Moving Platform/5(alpha_y) -> Integrator1/1
  Tx_L4/1 -> Moving Platform/22(Tx_L4)
  Tx_U2/1 -> Moving Platform/4(Tx_U2)
  Tx_L3/1 -> Moving Platform/19(Tx_L3)
  Moving Platform/1(ax) -> Integrator12/1
  wrap angle (Rad)/1(angle_out) -> MATLAB Function3/1(angle)
  Iy/1 -> Moving Platform/27(Iy)
  Integrator3/1 -> wrap angle (Rad)2/1(angle_in)
  Ty_L2/1 -> Moving Platform/17(Ty_L2)
  Ty_U4/1 -> Moving Platform/11(Ty_U4)
  Ty_U1/1 -> Moving Platform/2(Ty_U1)
  wrap angle (Rad)1/1(angle_out) -> MATLAB Function4/1(angle)
  Tz_U3/1 -> Moving Platform/9(Tz_U3)
  Moving Platform Transformation to Global/5(pitch) -> pitch/1, Derivative4/1
  Moving Platform/3(az) -> Integrator14/1
  MATLAB Function5/1(delta) -> Moving Platform Transformation to Global/4("roll ")
  Tx_L1/1 -> Moving Platform/13(Tx_L1)
  Iz/1 -> Moving Platform/28(Iz)
  Ty_U2/1 -> Moving Platform/5(Ty_U2)
  L/1 -> Moving Platform/32(L)
  Moving Platform Transformation to Global/2(Vby) -> Derivative1/1, Integrator6/1, Vy/1
  Tx_U4/1 -> Moving Platform/10(Tx_U4)
  Integrator/1 -> Integrator3/1
  Tz_L2/1 -> Moving Platform/18(Tz_L2)
  Tz_L1/1 -> Moving Platform/15(Tz_L1)
  Ty_L4/1 -> Moving Platform/23(Ty_L4)
  Integrator7/1 -> X/1
  H/1 -> Moving Platform/34(H)
  Ix/1 -> Moving Platform/26(Ix)
  Ty_L1/1 -> Moving Platform/14(Ty_L1)
  Tz_U2/1 -> Moving Platform/6(Tz_U2)
  mass/1 -> Moving Platform/25(m)
  Tz_L3/1 -> Moving Platform/21(Tz_L3)
  Tx_U1/1 -> Moving Platform/1(Tx_U1)
  Ty_U3/1 -> Moving Platform/8(Ty_U3)
  [gx] -> Delay/1
  [gy] -> Delay1/1
  Moving Platform Transformation to Global/7(gx) -> [gx]
  Moving Platform Transformation to Global/9(gz) -> [gz]
  Moving Platform Transformation to Global/8(gy) -> [gy]
  [gz] -> Delay2/1
  Delay2/1 -> IC/1
  Delay1/1 -> IC1/1
  Delay/1 -> IC2/1
  IC/1 -> Moving Platform/31(gz)
  IC1/1 -> Moving Platform/30(gy)
  Integrator12/1 -> Moving Platform Transformation to Global/1(Vx)
  Integrator13/1 -> Moving Platform Transformation to Global/2(Vy)
  Integrator14/1 -> Moving Platform Transformation to Global/3(Vz)
  Derivative/1 -> ax/1
  Derivative1/1 -> ay/1
  IC2/1 -> Moving Platform/29(gx)
  Integrator8/1 -> [Z], Z/1
  Moving Platform Transformation to Global/3(Vbz) -> Derivative3/1, Vz/1, Integrator8/1
  Derivative3/1 -> MATLAB Function/1(u)
  Derivative2/1 -> roll_dot/1
  Derivative4/1 -> pitch_dot/1
  Derivative5/1 -> yaw_dot/1
  Moving Platform Transformation to Global/10(rest) -> [rest]
  MATLAB Function/1(y) -> az/1
  [rest] -> MATLAB Function/2(rest)
  Delay3/1 -> IC3/1
  [Z] -> Delay3/1
  IC3/1 -> Moving Platform Transformation to Global/7(z)
  [rest] -> Subsystem1/1(rest)
  Subsystem1/2(A_init) -> Integrator8/3
  Subsystem1/1(A_rest) -> Integrator8/2
  Constant/1 -> Subsystem1/2(init)
  Vel_Manager/1(Vx_min) -> [Vx_min]
  Vel_Manager/3(Vz_min) -> [Vz_min]
  Vel_Manager/2(Vy_min) -> [Vy_min]
  Vel_Manager/4(Reste) -> [Reste]
  [Vx_min] -> Delay4/1
  [Vy_min] -> Delay5/1
  [Vz_min] -> Delay6/1
  [Reste] -> Moving Platform Transformation to Global/11(reste)
  Delay4/1 -> Moving Platform Transformation to Global/8(Vx_min)
  Delay5/1 -> Moving Platform Transformation to Global/9(Vy_min)
  Delay6/1 -> Moving Platform Transformation to Global/10(Vz_min)

== system cable_driven_parallel_robot2022/Actuators-CableTension-MovingPlatform/QuadRotor/QuadCopter Inputs ==
  W1 : Inport
  W2 : Inport  Port=2
  W3 : Inport  Port=3
  W4 : Inport  Port=4
  Tx : Inport  Port=5
  Ty : Inport  Port=6
  Tz : Inport  Port=7
  Constant : Constant  Value=QR_Iyy
  Constant1 : Constant  Value=QR_Izz
  Constant10 : Constant  Value=QR_Az
  Constant2 : Constant  Value=g
  Constant3 : Constant  Value=QR_l
  Constant4 : Constant  Value=QR_K
  Constant5 : Constant  Value=QR_b
  Constant6 : Constant  Value=QR_Ax
  Constant7 : Constant  Value=QR_Ay
  Constant8 : Constant  Value=QR_Ixx
  Constant9 : Constant  Value=QR_m
  Mux : Mux  Inputs=18
  Integrated Inputs : Outport
  wires:
  Constant5/1 -> Mux/8
  Constant6/1 -> Mux/9
  Constant9/1 -> Mux/1
  Constant3/1 -> Mux/6
  Constant10/1 -> Mux/11
  Constant7/1 -> Mux/10
  Constant4/1 -> Mux/7
  Mux/1 -> Integrated Inputs/1
  Constant8/1 -> Mux/3
  Constant/1 -> Mux/4
  Constant1/1 -> Mux/5
  Constant2/1 -> Mux/2
  Tx/1 -> Mux/16
  Ty/1 -> Mux/17
  Tz/1 -> Mux/18
  W1/1 -> Mux/12
  W2/1 -> Mux/13
  W3/1 -> Mux/14
  W4/1 -> Mux/15

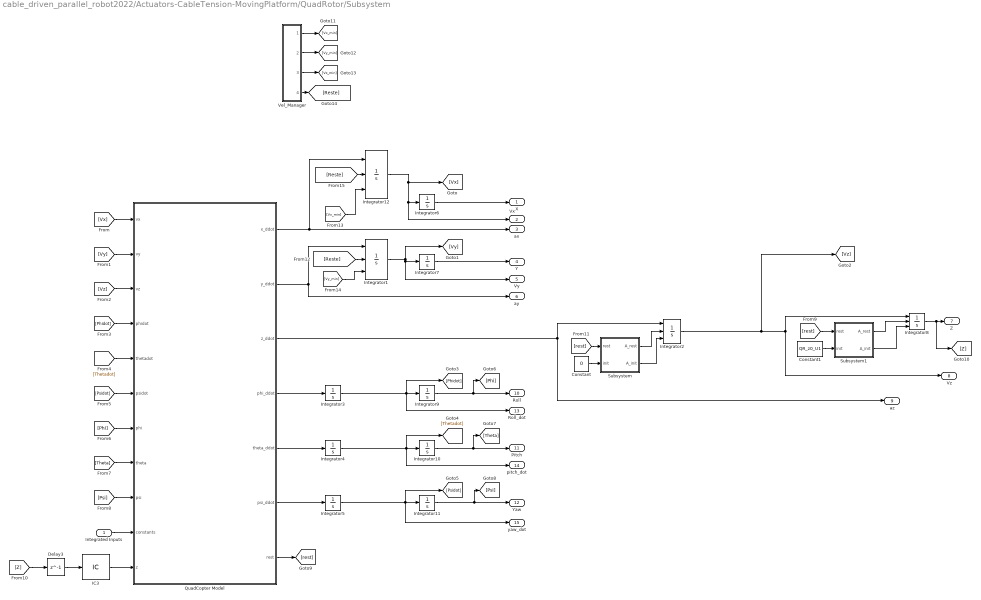
== system cable_driven_parallel_robot2022/Actuators-CableTension-MovingPlatform/QuadRotor/Subsystem ==
  Integrated Inputs : Inport
  Constant : Constant  Value=0
  Constant1 : Constant  Value=QR_z0_U1
  Delay3 : Delay  DelayLength=1
  IC3 : InitialCondition  Value=QR_z0_U1
  Integrator1 : Integrator  ExternalReset=rising  InitialConditionSource=external
  Integrator{3..5,9..11} (6 alike) : Integrator
  Integrator12 : Integrator  ExternalReset=rising  InitialConditionSource=external
  Integrator2 : Integrator  ExternalReset=rising  InitialConditionSource=external
  Integrator6 : Integrator  InitialCondition=QR_x0_U1
  Integrator7 : Integrator  InitialCondition=QR_y0_U1
  Integrator8 : Integrator  ExternalReset=rising  InitialConditionSource=external  InitialCondition=QR_z0_U1
  QuadCopter Model : MATLAB Function  TreatAsAtomicUnit=on
  Subsystem : Subsystem
  Subsystem1 : Subsystem
  Vel_Manager : Subsystem
  X : Outport
  Vx : Outport  Port=2
  ax : Outport  Port=3
  Y : Outport  Port=4
  Vy : Outport  Port=5
  ay : Outport  Port=6
  Z : Outport  Port=7
  Vz : Outport  Port=8
  az : Outport  Port=9
  Roll : Outport  Port=10
  Pitch : Outport  Port=11
  Yaw : Outport  Port=12
  Roll_dot : Outport  Port=13
  pitch_dot : Outport  Port=14
  yaw_dot : Outport  Port=15
  wires:
  QuadCopter Model/4(phi_ddot) -> Integrator3/1
  Integrator9/1 -> [Phi], Roll/1
  Integrator4/1 -> pitch_dot/1, [Thetadot], Integrator10/1
  QuadCopter Model/6(psi_ddot) -> Integrator5/1
  Integrator5/1 -> yaw_dot/1, [Psidot], Integrator11/1
  Integrator3/1 -> Roll_dot/1, [Phidot], Integrator9/1
  Integrator12/1 -> Vx/1, Integrator6/1, [Vx]
  Integrator10/1 -> [Theta], Pitch/1
  QuadCopter Model/5(theta_ddot) -> Integrator4/1
  QuadCopter Model/2(y_ddot) -> Integrator1/1, ay/1
  QuadCopter Model/1(x_ddot) -> Integrator12/1, ax/1
  Integrator11/1 -> [Psi], Yaw/1
  Integrator6/1 -> X/1
  Integrator7/1 -> Y/1
  Integrator8/1 -> [Z], Z/1
  Integrated Inputs/1 -> QuadCopter Model/10(constants)
  [Vx] -> QuadCopter Model/1(vx)
  [Vy] -> QuadCopter Model/2(vy)
  [Vz] -> QuadCopter Model/3(vz)
  [Phidot] -> QuadCopter Model/4(phidot)
  [Thetadot] -> QuadCopter Model/5(thetadot)
  [Psidot] -> QuadCopter Model/6(psidot)
  [Phi] -> QuadCopter Model/7(phi)
  [Theta] -> QuadCopter Model/8(theta)
  [Psi] -> QuadCopter Model/9(psi)
  Integrator1/1 -> [Vy], Vy/1, Integrator7/1
  Integrator2/1 -> [Vz], Vz/1, Integrator8/1
  QuadCopter Model/7(rest) -> [rest]
  [Z] -> Delay3/1
  Delay3/1 -> IC3/1
  IC3/1 -> QuadCopter Model/11(z)
  Constant/1 -> Subsystem/2(init)
  [rest] -> Subsystem/1(rest)
  Subsystem/1(A_rest) -> Integrator2/2
  Subsystem/2(A_init) -> Integrator2/3
  [rest] -> Subsystem1/1(rest)
  Subsystem1/1(A_rest) -> Integrator8/2
  Subsystem1/2(A_init) -> Integrator8/3
  Constant1/1 -> Subsystem1/2(init)
  [Vx_min] -> Integrator12/3
  [Reste] -> Integrator12/2
  Vel_Manager/1(Vx_min) -> [Vx_min]
  Vel_Manager/2(Vy_min) -> [Vy_min]
  Vel_Manager/3(Vz_min) -> [Vz_min]
  Vel_Manager/4(Reste) -> [Reste]
  [Reste] -> Integrator1/2
  [Vy_min] -> Integrator1/3
  QuadCopter Model/3(z_ddot) -> az/1, Integrator2/1

== system cable_driven_parallel_robot2022/Actuators-CableTension-MovingPlatform/QuadRotor1/QuadCopter Inputs ==
  W1 : Inport
  W2 : Inport  Port=2
  W3 : Inport  Port=3
  W4 : Inport  Port=4
  Tx : Inport  Port=5
  Ty : Inport  Port=6
  Tz : Inport  Port=7
  Constant : Constant  Value=QR_Iyy
  Constant1 : Constant  Value=QR_Izz
  Constant10 : Constant  Value=QR_Az
  Constant2 : Constant  Value=g
  Constant3 : Constant  Value=QR_l
  Constant4 : Constant  Value=QR_K
  Constant5 : Constant  Value=QR_b
  Constant6 : Constant  Value=QR_Ax
  Constant7 : Constant  Value=QR_Ay
  Constant8 : Constant  Value=QR_Ixx
  Constant9 : Constant  Value=QR_m
  Mux : Mux  Inputs=18
  Integrated Inputs : Outport
  wires:
  W4/1 -> Mux/15
  W3/1 -> Mux/14
  W2/1 -> Mux/13
  W1/1 -> Mux/12
  Tz/1 -> Mux/18
  Ty/1 -> Mux/17
  Tx/1 -> Mux/16
  Constant2/1 -> Mux/2
  Constant1/1 -> Mux/5
  Constant/1 -> Mux/4
  Constant8/1 -> Mux/3
  Mux/1 -> Integrated Inputs/1
  Constant4/1 -> Mux/7
  Constant7/1 -> Mux/10
  Constant10/1 -> Mux/11
  Constant3/1 -> Mux/6
  Constant9/1 -> Mux/1
  Constant6/1 -> Mux/9
  Constant5/1 -> Mux/8

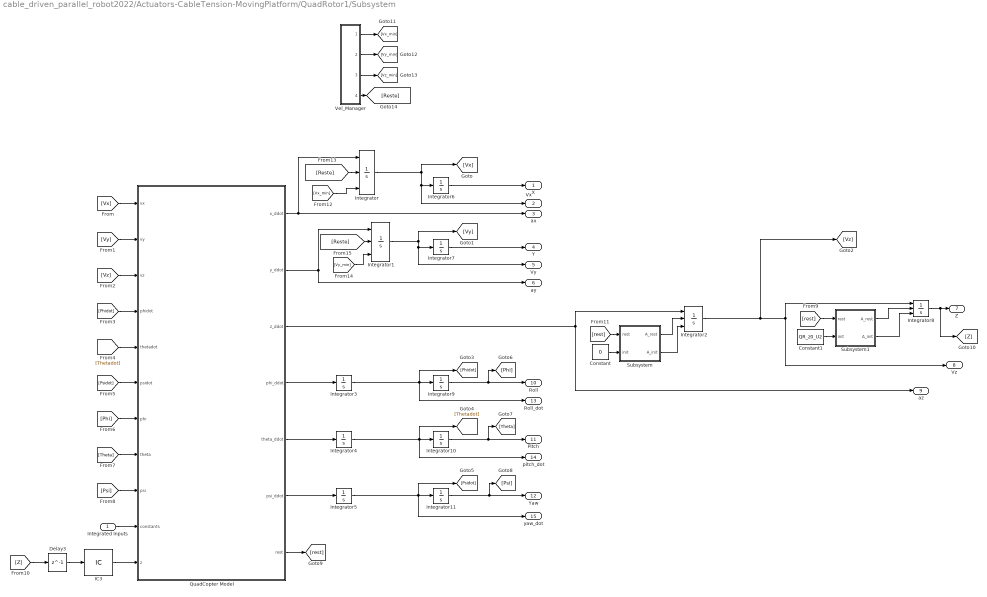
== system cable_driven_parallel_robot2022/Actuators-CableTension-MovingPlatform/QuadRotor1/Subsystem ==
  Integrated Inputs : Inport
  Constant : Constant  Value=0
  Constant1 : Constant  Value=QR_z0_U2
  Delay3 : Delay  DelayLength=1
  IC3 : InitialCondition  Value=QR_z0_U2
  Integrator : Integrator  ExternalReset=rising  InitialConditionSource=external
  Integrator1 : Integrator  ExternalReset=rising  InitialConditionSource=external
  Integrator{3..5,9..11} (6 alike) : Integrator
  Integrator2 : Integrator  ExternalReset=rising  InitialConditionSource=external
  Integrator6 : Integrator  InitialCondition=QR_x0_U2
  Integrator7 : Integrator  InitialCondition=QR_y0_U2
  Integrator8 : Integrator  ExternalReset=rising  InitialConditionSource=external  InitialCondition=QR_z0_U1
  QuadCopter Model : MATLAB Function  TreatAsAtomicUnit=on
  Subsystem : Subsystem
  Subsystem1 : Subsystem
  Vel_Manager : Subsystem
  X : Outport
  Vx : Outport  Port=2
  ax : Outport  Port=3
  Y : Outport  Port=4
  Vy : Outport  Port=5
  ay : Outport  Port=6
  Z : Outport  Port=7
  Vz : Outport  Port=8
  az : Outport  Port=9
  Roll : Outport  Port=10
  Pitch : Outport  Port=11
  Yaw : Outport  Port=12
  Roll_dot : Outport  Port=13
  pitch_dot : Outport  Port=14
  yaw_dot : Outport  Port=15
  wires:
  Constant1/1 -> Subsystem1/2(init)
  Subsystem1/2(A_init) -> Integrator8/3
  Subsystem1/1(A_rest) -> Integrator8/2
  [rest] -> Subsystem1/1(rest)
  Subsystem/2(A_init) -> Integrator2/3
  Subsystem/1(A_rest) -> Integrator2/2
  [rest] -> Subsystem/1(rest)
  Constant/1 -> Subsystem/2(init)
  IC3/1 -> QuadCopter Model/11(z)
  Delay3/1 -> IC3/1
  [Z] -> Delay3/1
  QuadCopter Model/7(rest) -> [rest]
  Integrator2/1 -> [Vz], Integrator8/1, Vz/1
  Integrator1/1 -> [Vy], Vy/1, Integrator7/1
  [Psi] -> QuadCopter Model/9(psi)
  [Theta] -> QuadCopter Model/8(theta)
  [Phi] -> QuadCopter Model/7(phi)
  [Psidot] -> QuadCopter Model/6(psidot)
  [Thetadot] -> QuadCopter Model/5(thetadot)
  [Phidot] -> QuadCopter Model/4(phidot)
  [Vz] -> QuadCopter Model/3(vz)
  [Vy] -> QuadCopter Model/2(vy)
  [Vx] -> QuadCopter Model/1(vx)
  Integrated Inputs/1 -> QuadCopter Model/10(constants)
  Integrator8/1 -> Z/1, [Z]
  Integrator7/1 -> Y/1
  Integrator6/1 -> X/1
  Integrator11/1 -> Yaw/1, [Psi]
  QuadCopter Model/1(x_ddot) -> ax/1, Integrator/1
  QuadCopter Model/2(y_ddot) -> Integrator1/1, ay/1
  QuadCopter Model/5(theta_ddot) -> Integrator4/1
  Integrator10/1 -> Pitch/1, [Theta]
  Integrator/1 -> Integrator6/1, Vx/1, [Vx]
  Integrator3/1 -> Integrator9/1, [Phidot], Roll_dot/1
  Integrator5/1 -> Integrator11/1, [Psidot], yaw_dot/1
  QuadCopter Model/6(psi_ddot) -> Integrator5/1
  Integrator4/1 -> Integrator10/1, [Thetadot], pitch_dot/1
  Integrator9/1 -> Roll/1, [Phi]
  QuadCopter Model/4(phi_ddot) -> Integrator3/1
  Vel_Manager/3(Vz_min) -> [Vz_min]
  Vel_Manager/1(Vx_min) -> [Vx_min]
  Vel_Manager/4(Reste) -> [Reste]
  Vel_Manager/2(Vy_min) -> [Vy_min]
  [Vx_min] -> Integrator/3
  [Reste] -> Integrator/2
  [Vy_min] -> Integrator1/3
  [Reste] -> Integrator1/2
  QuadCopter Model/3(z_ddot) -> Integrator2/1, az/1

== system cable_driven_parallel_robot2022/Actuators-CableTension-MovingPlatform/QuadRotor2/QuadCopter Inputs ==
  W1 : Inport
  W2 : Inport  Port=2
  W3 : Inport  Port=3
  W4 : Inport  Port=4
  Tx : Inport  Port=5
  Ty : Inport  Port=6
  Tz : Inport  Port=7
  Constant : Constant  Value=QR_Iyy
  Constant1 : Constant  Value=QR_Izz
  Constant10 : Constant  Value=QR_Az
  Constant2 : Constant  Value=g
  Constant3 : Constant  Value=QR_l
  Constant4 : Constant  Value=QR_K
  Constant5 : Constant  Value=QR_b
  Constant6 : Constant  Value=QR_Ax
  Constant7 : Constant  Value=QR_Ay
  Constant8 : Constant  Value=QR_Ixx
  Constant9 : Constant  Value=QR_m
  Mux : Mux  Inputs=18
  Integrated Inputs : Outport
  wires:
  Constant5/1 -> Mux/8
  Constant6/1 -> Mux/9
  Constant9/1 -> Mux/1
  Constant3/1 -> Mux/6
  Constant10/1 -> Mux/11
  Constant7/1 -> Mux/10
  Constant4/1 -> Mux/7
  Mux/1 -> Integrated Inputs/1
  Constant8/1 -> Mux/3
  Constant/1 -> Mux/4
  Constant1/1 -> Mux/5
  Constant2/1 -> Mux/2
  Tx/1 -> Mux/16
  Ty/1 -> Mux/17
  Tz/1 -> Mux/18
  W1/1 -> Mux/12
  W2/1 -> Mux/13
  W3/1 -> Mux/14
  W4/1 -> Mux/15
